simulink model "tb_q_current_control"  (R2025b)
settings: Solver=VariableStepAuto  StartTime=0.0  StopTime=0.004  RelTol=1e-3
undefined symbols (not defined in the file or in its folder): control, motor
settings Model: Creator=semih  LastModifiedBy=semih

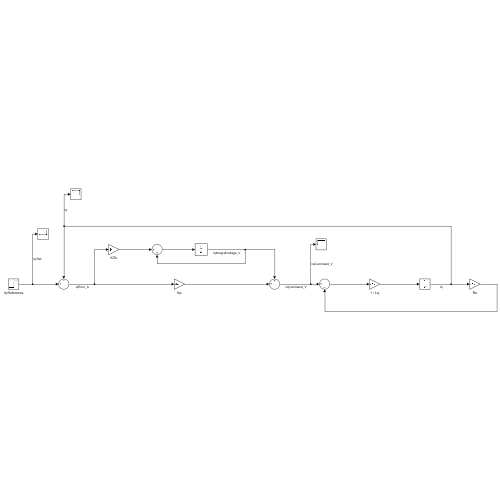
[thumbnail: Simulink's stored preview of the top-level diagram]
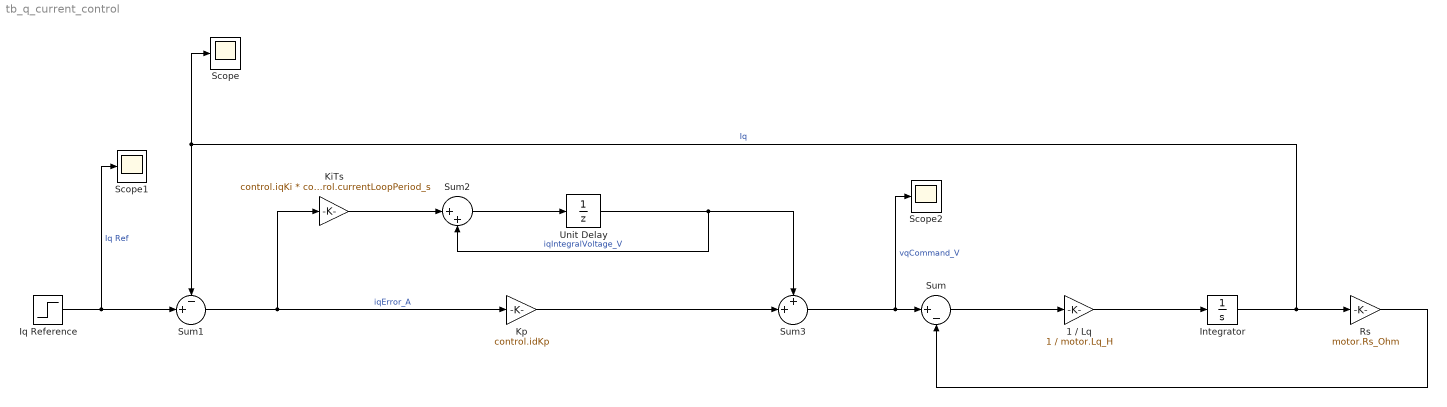
== system tb_q_current_control ==
  1 / Lq : Gain  Gain=1 / motor.Lq_H
  Integrator : Integrator  InitialCondition=motor.iq0_A
  Iq Reference : Step  Time=0.001  After=2  SampleTime=0
  KiTs : Gain  Gain=control.iqKi * control.currentLoopPeriod_s
  Kp : Gain  Gain=control.idKp
  Rs : Gain  Gain=motor.Rs_Ohm
  Scope : Scope
      settings: ActiveDisplayYMinimum=-0.25501614631792935  ActiveDisplayYMaximum=2.2951453168613645
  Scope1 : Scope
      settings: ActiveDisplayYMinimum=-0.24999999999999994  ActiveDisplayYMaximum=2.25
  Scope2 : Scope
      settings: ActiveDisplayYMinimum=1.6049299584249686  ActiveDisplayYMaximum=3.7656681894500852  DataLoggingVariableName=ScopeData2
  Sum : Sum  Inputs=|+-
  Sum1 : Sum  Inputs=-+|
  Sum2 : Sum  Inputs=|++
  Sum3 : Sum  Inputs=++|
  Unit Delay : UnitDelay  SampleTime=control.currentLoopPeriod_s  HasFrameUpgradeWarning=on
  wires:
  Integrator/1 -> Scope/1, Sum1/1, Rs/1  "Iq"
  1 / Lq/1 -> Integrator/1
  Sum/1 -> 1 / Lq/1
  Rs/1 -> Sum/2
  Sum1/1 -> KiTs/1, Kp/1  "iqError_A"
  KiTs/1 -> Sum2/1
  Sum2/1 -> Unit Delay/1
  Unit Delay/1 -> Sum3/1, Sum2/2  "iqIntegralVoltage_V"
  Kp/1 -> Sum3/2
  Sum3/1 -> Scope2/1, Sum/1  "vqCommand_V"
  Iq Reference/1 -> Scope1/1, Sum1/2  "Iq Ref"
